simulink model "DSP"  (R2024b)
settings: Solver=FixedStepDiscrete  StartTime=0.0  StopTime=25  MaxStep=1e-6  RelTol=1e-12  AbsTol=1e-3
libraries: dspvision x4, dspxfrm3 x3, dspstat3 x2, dspsnks4 x1, dspsigops x1
settings Model: Creator=chira  LastModifiedBy=Hp
settings SolverCC: ZeroCrossControl=DisableAll  ZeroCrossAlgorithm=Adaptive
settings ModelReferenceCC: EnableRefExpFcnMdlSchedulingChecks=on
settings RTWCC: GPUComputeCapability=3.5

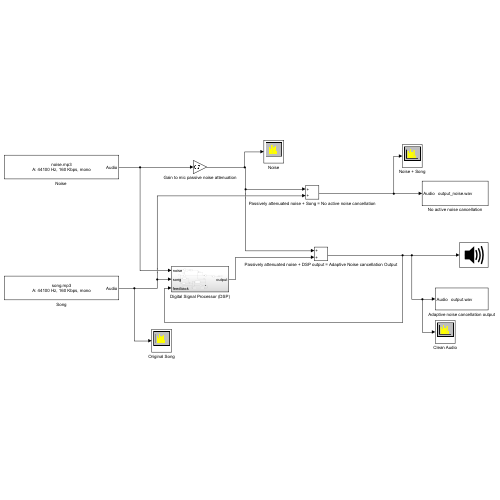
[thumbnail: Simulink's stored preview of the top-level diagram]
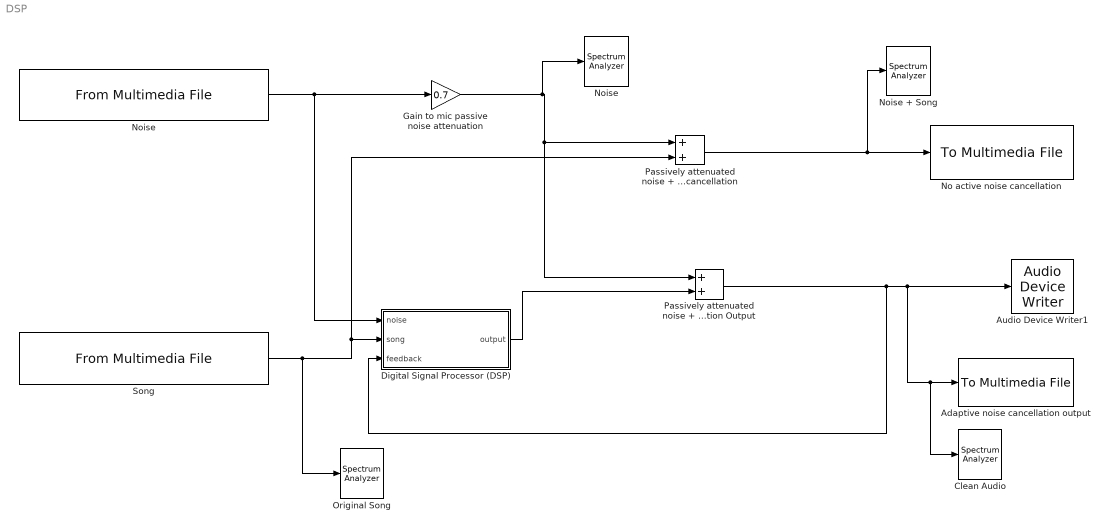
== system DSP ==
  Adaptive noise cancellation output : dspvision/To Multimedia File  outputFilename=output.wav  streamSelection=Audio only  videoCompressor=None (uncompressed)  audioCompressor=None (uncompressed)  imagePorts=Separate color signals  fileType=WAV  audioDatatype=16-bit integer  fourcc=RGB  audioBitRate=128  audioQuality=75  videoQuality=75  mj2000CompFactor=10
  Audio Device Writer1 : dspsnks4/Audio Device Writer  Driver=DirectSound  Device=Default  InheritSampleRate=on  SampleRate=44100  BitDepth=16-bit integer  BufferSize=4096  NumBuffers=10  DefaultOutputChannelMapping=on  OutputChannelMapping=1:2  OutputNumUnderrunSamples=off  DriverIdx=1  DeviceWarnFlag=''
  Clean Audio : SpectrumAnalyzer  WindowPosition=[769.000000,49.000000,766.000000,376.000000,]  Visible=on  ScopeFrameLocation=window  SampleRateSource=Property  SampleRate=44.1e3  PlotAsTwoSidedSpectrum=off  FrequencyScale=Log  FrequencySpan=Start and stop frequencies  StartFrequency=20  StopFrequency=20e3  AveragingMethod=Exponential  YLimits=[-108.4777399,27.69652832]  AllowFFTLengthLessThanSamplesPerUpdate=on
  Digital Signal Processor (DSP) : Subsystem
  Gain to mic passive noise attenuation : Gain  Gain=0.7
  No active noise cancellation : dspvision/To Multimedia File  outputFilename=output_noise.wav  streamSelection=Audio only  videoCompressor=None (uncompressed)  audioCompressor=None (uncompressed)  imagePorts=Separate color signals  fileType=WAV  audioDatatype=16-bit integer  fourcc=RGB  audioBitRate=128  audioQuality=75  videoQuality=75  mj2000CompFactor=10
  Noise : SpectrumAnalyzer  WindowPosition=[769.000000,457.000000,766.000000,376.000000,]  Visible=on  ScopeFrameLocation=window  SampleRateSource=Property  SampleRate=44.1e3  PlotAsTwoSidedSpectrum=off  FrequencyScale=Log  FrequencySpan=Start and stop frequencies  StartFrequency=20  StopFrequency=20e3  AveragingMethod=Exponential  YLimits=[-110.41018095,15.77282431]  AllowFFTLengthLessThanSamplesPerUpdate=on
  "Noise " : dspvision/From Multimedia File  inputFilename=D:\PROJECTS\DSP\original\mono\noise.mp3  readRange=[1 Inf]  loop=on  numPlays=inf  outputStreams=Audio only  videoDataType=single  audioDataType=double  inheritSampleTime=on  userDefinedSampleTime=1/30  noAudioOutput=off  isIntensityVideo=off  fourcc=RGB  colorVideoFormat=Separate color signals  outputEOF=off  dataOrg=Column-major  audioFrameSize=1024  computeAudioFrameSize=off  outSamplingMode=Sample based
  Noise + Song : SpectrumAnalyzer  WindowPosition=[1.000000,49.000000,766.000000,376.000000,]  Visible=on  ScopeFrameLocation=window  SampleRateSource=Property  SampleRate=44.1e3  PlotAsTwoSidedSpectrum=off  FrequencyScale=Log  FrequencySpan=Start and stop frequencies  StartFrequency=20  StopFrequency=20e3  AveragingMethod=Exponential  YLimits=[-110.01206798,27.9117373]  AllowFFTLengthLessThanSamplesPerUpdate=on
  Original Song : SpectrumAnalyzer  WindowPosition=[1.000000,457.000000,766.000000,376.000000,]  Visible=on  ScopeFrameLocation=window  SampleRateSource=Property  SampleRate=44.1e3  PlotAsTwoSidedSpectrum=off  FrequencyScale=Log  FrequencySpan=Start and stop frequencies  StartFrequency=20  StopFrequency=20e3  AveragingMethod=Exponential  YLimits=[-118.04064686,28.65576591]  AllowFFTLengthLessThanSamplesPerUpdate=on
  Passively attenuated noise + DSP output = Adaptive Noise cancellation Output : Sum
  Passively attenuated noise + Song = No active noise cancellation : Sum
  Song : dspvision/From Multimedia File  inputFilename=D:\PROJECTS\DSP\original\mono\song.mp3  readRange=[1 Inf]  loop=on  numPlays=inf  outputStreams=Audio only  videoDataType=single  audioDataType=double  inheritSampleTime=on  userDefinedSampleTime=1/30  noAudioOutput=off  isIntensityVideo=off  fourcc=RGB  colorVideoFormat=Separate color signals  outputEOF=off  dataOrg=Column-major  audioFrameSize=1024  computeAudioFrameSize=off  outSamplingMode=Sample based
  wires:
  "Noise "/1 -> Digital Signal Processor (DSP)/1(noise), Gain to mic passive noise attenuation/1
  Gain to mic passive noise attenuation/1 -> Noise/1, Passively attenuated noise + Song = No active noise cancellation/1, Passively attenuated noise + DSP output = Adaptive Noise cancellation Output/1
  Passively attenuated noise + DSP output = Adaptive Noise cancellation Output/1 -> Clean Audio/1, Adaptive noise cancellation output/1, Audio Device Writer1/1, Digital Signal Processor (DSP)/3(feedback)
  Song/1 -> Original Song/1, Passively attenuated noise + Song = No active noise cancellation/2, Digital Signal Processor (DSP)/2(song)
  Digital Signal Processor (DSP)/1(output) -> Passively attenuated noise + DSP output = Adaptive Noise cancellation Output/2
  Passively attenuated noise + Song = No active noise cancellation/1 -> Noise + Song/1, No active noise cancellation/1

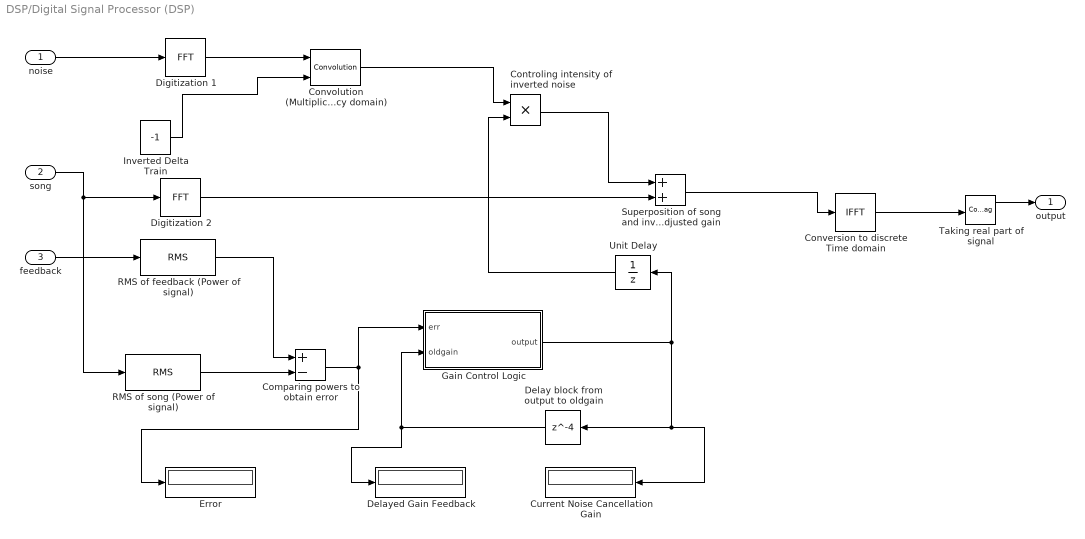
== system DSP/Digital Signal Processor (DSP) ==
  noise : Inport
  song : Inport  Port=2
  feedback : Inport  Port=3
  Comparing powers to obtain error : Sum  Inputs=+-
  Controling intensity of inverted noise : Product
  Conversion to discrete Time domain : dspxfrm3/IFFT  FFTImplementation=Auto  CompMethod=Table lookup  TableOpt=NEW  TableOptActive=Speed  BitRevOrder=off  cs_in=off  Normalize=on  InheritFFTLength=on  FFTLength=64  WrapInput=on  mode=Complex  outSamplingMode=Sample based  roundingMode=Floor  overflowMode=off  firstCoeffDataTypeStr=Inherit: Same word length as input  firstCoeffLastDataTypeStr=Inherit: Same word length as input  outputMin=[]  outputMax=[]
  Convolution (Multiplication in time domain is convolution in frequency domain) : dspsigops/Convolution  domain=Time  roundingMode=Floor  overflowMode=off  outputDataTypeStr=Inherit: Same as accumulator  outputMin=[]  outputMax=[]  outputLastDataTypeStr=Inherit: Same as accumulator
  Current Noise Cancellation Gain : Display
  Delay block from output to oldgain : Delay  DelayLength=4
  Delayed Gain Feedback : Display
  Digitization 1 : dspxfrm3/FFT  FFTImplementation=Auto  CompMethod=Table lookup  TableOpt=NEW  TableOptActive=Speed  BitRevOrder=off  Normalize=off  InheritFFTLength=on  FFTLength=64  WrapInput=on  roundingMode=Floor  overflowMode=off  firstCoeffDataTypeStr=Inherit: Same word length as input  firstCoeffLastDataTypeStr=Inherit: Same word length as input  outputMin=[]  outputMax=[]
  Digitization 2 : dspxfrm3/FFT  FFTImplementation=Auto  CompMethod=Table lookup  TableOpt=NEW  TableOptActive=Speed  BitRevOrder=off  Normalize=off  InheritFFTLength=on  FFTLength=64  WrapInput=on  roundingMode=Floor  overflowMode=off  firstCoeffDataTypeStr=Inherit: Same word length as input  firstCoeffLastDataTypeStr=Inherit: Same word length as input  outputMin=[]  outputMax=[]
  Error : Display
  Gain Control Logic : MATLAB Function  TreatAsAtomicUnit=on
  Inverted Delta Train : Constant  Value=-1  VectorParams1D=off
  RMS of feedback (Power of signal) : dspstat3/RMS  run=off  directionMode=Each column  dimension=1  InputProcessing=Columns as channels (frame based)  reset_popup=None
  RMS of song (Power of signal) : dspstat3/RMS  run=off  directionMode=Each column  dimension=1  InputProcessing=Columns as channels (frame based)  reset_popup=None
  Superposition of song and inverted noise with adjusted gain : Sum
  Taking real part of signal : ComplexToRealImag
  Unit Delay : UnitDelay  SampleTime=-1  HasFrameUpgradeWarning=on
  output : Outport
  wires:
  song/1 -> Digitization 2/1, RMS of song (Power of signal)/1
  Digitization 2/1 -> Superposition of song and inverted noise with adjusted gain/2
  noise/1 -> Digitization 1/1
  Digitization 1/1 -> Convolution (Multiplication in time domain is convolution in frequency domain)/1
  Inverted Delta Train/1 -> Convolution (Multiplication in time domain is convolution in frequency domain)/2
  Conversion to discrete Time domain/1 -> Taking real part of signal/1
  Taking real part of signal/1 -> output/1
  Superposition of song and inverted noise with adjusted gain/1 -> Conversion to discrete Time domain/1
  feedback/1 -> RMS of feedback (Power of signal)/1
  Gain Control Logic/1(output) -> Unit Delay/1, Current Noise Cancellation Gain/1, Delay block from output to oldgain/1
  Controling intensity of inverted noise/1 -> Superposition of song and inverted noise with adjusted gain/1
  Convolution (Multiplication in time domain is convolution in frequency domain)/1 -> Controling intensity of inverted noise/1
  RMS of feedback (Power of signal)/1 -> Comparing powers to obtain error/1
  RMS of song (Power of signal)/1 -> Comparing powers to obtain error/2
  Comparing powers to obtain error/1 -> Gain Control Logic/1(err), Error/1
  Delay block from output to oldgain/1 -> Delayed Gain Feedback/1, Gain Control Logic/2(oldgain)
  Unit Delay/1 -> Controling intensity of inverted noise/2

== matlab function DSP/Digital Signal Processor (DSP)/Gain Control Logic ==
  data: err input; output output; oldgain input
function output  = fcn(err,oldgain)
req_err = 0.0001;


if((req_err<=err))
output=oldgain+0.005;
else
output=oldgain;    
end
end
